simulink model "sfLeaveError"  (R2025b)
settings: Solver=VariableStepAuto  StartTime=0.0  StopTime=10.0  RelTol=1e-3
settings Model: Creator=The MathWorks, Inc.  LastModifiedBy=The MathWorks, Inc.

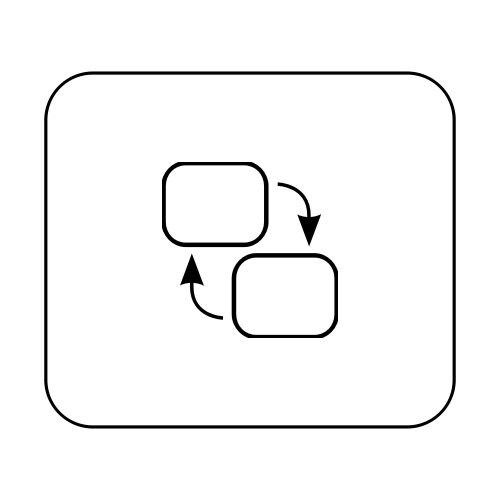
[thumbnail: Simulink's stored preview of the top-level diagram]
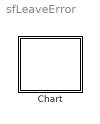
== system sfLeaveError ==
  Chart : Stateflow chart  TreatAsAtomicUnit=on

== stateflow chart sfLeaveError/Chart ==
  state A
    on every(5,tick): leave;
  state B
  (default) -> A
  A -> B : leave
  B -> A
  events: leave local FUNCTION_CALL_EVENT
